simulink model "NBMS_MosfetSeq"  (R2026b)
settings: Solver=FixedStepDiscrete  StopTime=25  FixedStep=0.1
undefined symbols (not defined in the file): CAL_MOSFET_DISENG_THRSH, CAL_MOSFET_FEEDBACK, MosfetTime
settings Model: Creator=hp  LastModifiedBy=rathi
settings OptimizationCC: DefaultParameterBehavior=Inlined  DifferentSizesBufferReuse=on  EfficientTunableParamExpr=on  EnhancedBackFolding=on  OptimizationCustomize=off  OptimizeBlockOrder=speed  PassReuseOutputArgsAs=Individual arguments  RemoveInternalMemoryZeroInit=on  RemoveRootLevelIOMemoryZeroInit=on
settings DebuggingCC: ParameterTunabilityLossMsg=error
settings SFSimCC: MATLABDynamicMemAlloc=off
settings RTWCC: Description=Embedded Coder  GenCodeOnly=on  PackageGeneratedCodeAndArtifacts=on  SystemTargetFile=ert.tlc  TemplateMakefile=ert_default_tmf
settings CodeAppCC: ForceParamTrailComments=on  IgnoreCustomStorageClasses=off  InsertBlockDesc=on  OperatorAnnotations=on  SFDataObjDesc=on  SimulinkDataObjDesc=on
settings ERTTargetCC: DynamicArrayContainerType=coder::array  GenerateSampleERTMain=on
settings ConfigComp: DVDefectChecker=on  DVDetectOutOfBounds=on  DVHarnessSource=Signal Editor  DVModelReferenceHarness=on  DVTestSuiteOptimization=Auto

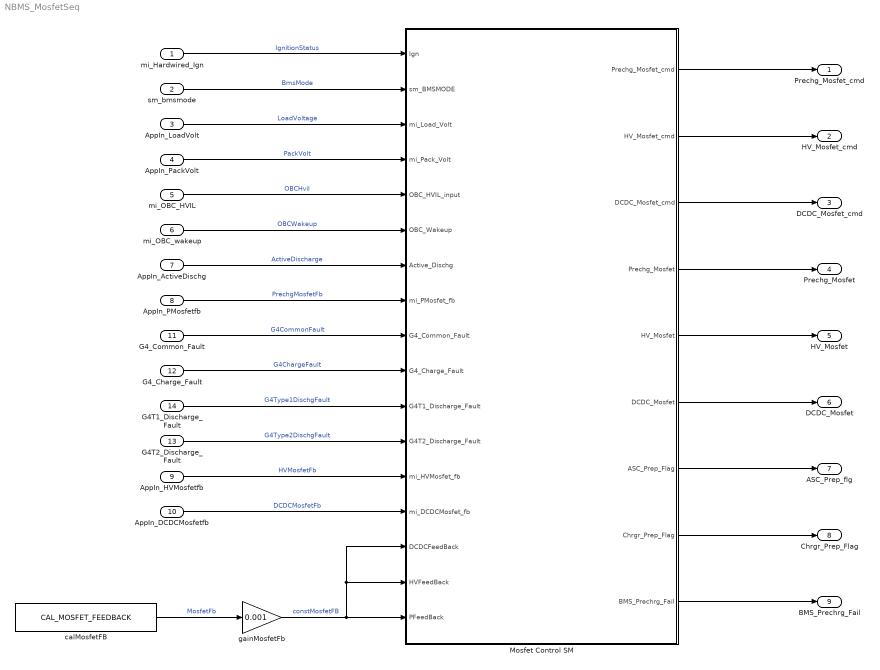
== system NBMS_MosfetSeq ==
  mi_Hardwired_Ign : Inport  OutDataTypeStr=boolean
  sm_bmsmode : Inport  Port=2  OutDataTypeStr=Enum: BMS_MODE_E
  AppIn_LoadVolt : Inport  Port=3  OutDataTypeStr=double
  AppIn_PackVolt : Inport  Port=4  OutDataTypeStr=double
  mi_OBC_HVIL : Inport  Port=5  OutDataTypeStr=boolean
  mi_OBC_wakeup : Inport  Port=6  OutDataTypeStr=Enum: OBC_E
  AppIn_ActiveDischg : Inport  Port=7  OutDataTypeStr=Enum: Active_DisChrg_E
  AppIn_PMosfetfb : Inport  Port=8  OutDataTypeStr=boolean
  AppIn_HVMosfetfb : Inport  Port=9  OutDataTypeStr=boolean
  AppIn_DCDCMosfetfb : Inport  Port=10  OutDataTypeStr=boolean
  G4_Common_Fault : Inport  Port=11  OutDataTypeStr=boolean
  G4_Charge_Fault : Inport  Port=12  OutDataTypeStr=boolean
  G4T2_Discharge_Fault : Inport  Port=13  OutDataTypeStr=boolean
  G4T1_Discharge_Fault : Inport  Port=14  OutDataTypeStr=boolean
  Mosfet Control SM : Stateflow chart  TreatAsAtomicUnit=on
      settings: PortSchema="{\"entries\":[{\"content\":{\"sides\":[{\"content\":{\"connectorIds\":[\"In1\",\"In2\",\"In3\",\"In4\",\"In5\",\"In6\",\"In7\",\"In13\",\"In14\",\"In15\",\"In16\",\"In17\",\"In12\",\"In11\",\"In8\",\"In9\",\"In10\"]},\"type\":\"ConnectorPlacement.EquallySpacedRectSide\",\"uuid\":\"999ebbd4-8031-46c1-80ce-b4c49c4d20a6\"},{\"content\":{\"connectorIds\":[\"Out1\",\"Out2\",\"Out3\",\"Out4\",\"Out5\",\"Out6\",\"Out7\",\"Out8\",\"Out9\"],\"side\":\"RIGHT\"},\"type\":\"ConnectorPlacement.EquallySpacedRectSide\",\"uuid\":\"fef7eb13-12a9-441d-9d81-95e69bfbb711\"},{\"content\":{\"side\":\"TOP\"},\"type\":\"ConnectorPlacement.EquallySpacedRectSide\",\"uuid\":\"5f60749b-759b-4b11-83fc-c9d02330dc93\"}]},\"type\":\"ConnectorPlacement.EquallySpacedConnector\",\"uuid\":\"de7edef1-d0c8-483b-a7d7-5a99a93b68ab\"}],\"packageUris\":[\"http://schema.mathworks.com/mf0/Connector/R2020b\"],\"version\":\"1.0\"}"
  calMosfetFB : Constant  Value=CAL_MOSFET_FEEDBACK
  gainMosfetFb : Gain  Gain=0.001  OutDataTypeStr=double
  Prechg_Mosfet_cmd : Outport  OutDataTypeStr=boolean
  HV_Mosfet_cmd : Outport  Port=2  OutDataTypeStr=boolean
  DCDC_Mosfet_cmd : Outport  Port=3  OutDataTypeStr=boolean
  Prechg_Mosfet : Outport  Port=4  OutDataTypeStr=Enum: BMS_PMosfet_STS_E
  HV_Mosfet : Outport  Port=5  OutDataTypeStr=Enum: BMS_HVMosfet_STS_E
  DCDC_Mosfet : Outport  Port=6  OutDataTypeStr=Enum: BMS_DCDCMosfet_STS_E
  ASC_Prep_flg : Outport  Port=7  OutDataTypeStr=boolean
  Chrgr_Prep_Flag : Outport  Port=8  OutDataTypeStr=boolean
  BMS_Prechrg_Fail : Outport  Port=9  OutDataTypeStr=boolean
  wires:
  mi_Hardwired_Ign/1 -> Mosfet Control SM/1(Ign)  "IgnitionStatus"
  sm_bmsmode/1 -> Mosfet Control SM/2(sm_BMSMODE)  "BmsMode"
  AppIn_LoadVolt/1 -> Mosfet Control SM/3(mi_Load_Volt)  "LoadVoltage"
  AppIn_PackVolt/1 -> Mosfet Control SM/4(mi_Pack_Volt)  "PackVolt"
  mi_OBC_HVIL/1 -> Mosfet Control SM/5(OBC_HVIL_input)  "OBCHvil"
  mi_OBC_wakeup/1 -> Mosfet Control SM/6(OBC_Wakeup)  "OBCWakeup"
  AppIn_ActiveDischg/1 -> Mosfet Control SM/7(Active_Dischg)  "ActiveDischarge"
  Mosfet Control SM/3(DCDC_Mosfet_cmd) -> DCDC_Mosfet_cmd/1
  Mosfet Control SM/2(HV_Mosfet_cmd) -> HV_Mosfet_cmd/1
  Mosfet Control SM/1(Prechg_Mosfet_cmd) -> Prechg_Mosfet_cmd/1
  Mosfet Control SM/4(Prechg_Mosfet) -> Prechg_Mosfet/1
  Mosfet Control SM/5(HV_Mosfet) -> HV_Mosfet/1
  Mosfet Control SM/6(DCDC_Mosfet) -> DCDC_Mosfet/1
  Mosfet Control SM/7(ASC_Prep_Flag) -> ASC_Prep_flg/1
  calMosfetFB/1 -> gainMosfetFb/1  "MosfetFb"
  gainMosfetFb/1 -> Mosfet Control SM/8(DCDCFeedBack), Mosfet Control SM/9(HVFeedBack), Mosfet Control SM/10(PFeedBack)  "constMosfetFB"
  AppIn_PMosfetfb/1 -> Mosfet Control SM/13(mi_PMosfet_fb)  "PrechgMosfetFb"
  AppIn_HVMosfetfb/1 -> Mosfet Control SM/12(mi_HVMosfet_fb)  "HVMosfetFb"
  AppIn_DCDCMosfetfb/1 -> Mosfet Control SM/11(mi_DCDCMosfet_fb)  "DCDCMosfetFb"
  G4_Common_Fault/1 -> Mosfet Control SM/14(G4_Common_Fault)  "G4CommonFault"
  G4_Charge_Fault/1 -> Mosfet Control SM/15(G4_Charge_Fault)  "G4ChargeFault"
  G4T2_Discharge_Fault/1 -> Mosfet Control SM/17(G4T2_Discharge_Fault)  "G4Type2DischgFault"
  G4T1_Discharge_Fault/1 -> Mosfet Control SM/16(G4T1_Discharge_Fault)  "G4Type1DischgFault"
  Mosfet Control SM/8(Chrgr_Prep_Flag) -> Chrgr_Prep_Flag/1
  Mosfet Control SM/9(BMS_Prechrg_Fail) -> BMS_Prechrg_Fail/1

== stateflow chart NBMS_MosfetSeq/Mosfet Control SM ==
  state DEFAULT
    state DEF
    state STANDBY
      state DEFAULT
        HV_Mosfet_cmd = false;
      state OpenHVMosfet
        HV_Mosfet = BMS_HVMosfet_STS_E.HV_DISCONNECTED;
      state OpenDCDCMosfet
        en:
        DCDC_Mosfet_cmd = false;
        DCDC_Mosfet = BMS_DCDCMosfet_STS_E.DCDC_DISCONNECTED;
      (default) -> DEFAULT.STANDBY.DEFAULT : {NA = false;}
      DEFAULT.STANDBY.DEFAULT -> DEFAULT.STANDBY.OpenHVMosfet : [duration(mi_HVMosfet_fb==0)>=HVFeedBack]
      DEFAULT.STANDBY.OpenHVMosfet -> DEFAULT.STANDBY.OpenDCDCMosfet : [Active_Dischg == Active_DisChrg_E.Completed || ...
          | sm_BMSMODE == BMS_MODE_E.BMS_SLEEP]
    state No_Action
      NA = true;
      state CloseDCDC
        DCDC_Mosfet_cmd = true;
        DCDC_Mosfet = BMS_DCDCMosfet_STS_E.DCDC_CONNECTED;
      state OpenDCDC
        DCDC_Mosfet_cmd = false;
        DCDC_Mosfet = BMS_DCDCMosfet_STS_E.DCDC_DISCONNECTED;
      (default) -> DEFAULT.No_Action.CloseDCDC
      DEFAULT.No_Action.CloseDCDC -> DEFAULT.No_Action.OpenDCDC : [sm_BMSMODE == BMS_MODE_E.BMS_CHARGE && Ign == false]
      DEFAULT.No_Action.OpenDCDC -> DEFAULT.No_Action.CloseDCDC : [Ign == true]
    state G4CommonFault
      state OnFaultDetection
        state OpenHVMosfet
          en:
          Prechg_Mosfet = BMS_PMosfet_STS_E.PDISCONNECTED;
          HV_Mosfet = BMS_HVMosfet_STS_E.HV_DISCONNECTED;
          Prechg_Mosfet_cmd = false;
          HV_Mosfet_cmd = false;
        state Def
          en:
          count1 = 0;
          du:
          count1 = count1 + 100;
        (default) -> DEFAULT.G4CommonFault.OnFaultDetection.Def
        DEFAULT.G4CommonFault.OnFaultDetection.Def -> DEFAULT.G4CommonFault.OnFaultDetection.OpenHVMosfet : [count1>=CAL_MOSFET_DISENG_THRSH]
            | {NA = false; Chrgr_Prep_Flag = false; ASC_Prep_Flag = false;}
      state BMS_Sleep
        en:
        Prechg_Mosfet = BMS_PMosfet_STS_E.PDISCONNECTED;
        HV_Mosfet = BMS_HVMosfet_STS_E.HV_DISCONNECTED;
        DCDC_Mosfet = BMS_DCDCMosfet_STS_E.DCDC_DISCONNECTED;
        Prechg_Mosfet_cmd = false;
        HV_Mosfet_cmd = false;
        DCDC_Mosfet_cmd = false;
        BMS_Prechrg_Fail = false;
      (default) -> DEFAULT.G4CommonFault.OnFaultDetection
      DEFAULT.G4CommonFault.OnFaultDetection -> DEFAULT.G4CommonFault.BMS_Sleep : [(sm_BMSMODE == BMS_MODE_E.BMS_FAULT && Ign == false && ...
          | Active_Dischg == Active_DisChrg_E.Completed) || ...
          | sm_BMSMODE == BMS_MODE_E.BMS_SLEEP]
    state G4Typ1DischgFault
      state OnFaultDetection
        state OpenHVMosfet
          en:
          Prechg_Mosfet = BMS_PMosfet_STS_E.PDISCONNECTED;
          HV_Mosfet = BMS_HVMosfet_STS_E.HV_DISCONNECTED;
          Prechg_Mosfet_cmd = false;
          HV_Mosfet_cmd = false;
        state Def
          en:
          count = 0;
          du:
          count = count + 100;
        (default) -> DEFAULT.G4Typ1DischgFault.OnFaultDetection.Def
        DEFAULT.G4Typ1DischgFault.OnFaultDetection.Def -> DEFAULT.G4Typ1DischgFault.OnFaultDetection.OpenHVMosfet : [count>=CAL_MOSFET_DISENG_THRSH]
            | {NA = false; ASC_Prep_Flag = false;}
      state BMS_Sleep
        en:
        Prechg_Mosfet = BMS_PMosfet_STS_E.PDISCONNECTED;
        HV_Mosfet = BMS_HVMosfet_STS_E.HV_DISCONNECTED;
        DCDC_Mosfet = BMS_DCDCMosfet_STS_E.DCDC_DISCONNECTED;
        Prechg_Mosfet_cmd = false;
        HV_Mosfet_cmd = false;
        DCDC_Mosfet_cmd = false;
        BMS_Prechrg_Fail = false;
      (default) -> DEFAULT.G4Typ1DischgFault.OnFaultDetection
      DEFAULT.G4Typ1DischgFault.OnFaultDetection -> DEFAULT.G4Typ1DischgFault.BMS_Sleep : [(sm_BMSMODE == BMS_MODE_E.BMS_FAULT && Ign == false && ...
          | Active_Dischg == Active_DisChrg_E.Completed) || ...
          | sm_BMSMODE == BMS_MODE_E.BMS_SLEEP]
    state G4Typ2DischgFault
      state OnFaultDetection
        state OpenHVMosfet
          en:
          Prechg_Mosfet = BMS_PMosfet_STS_E.PDISCONNECTED;
          HV_Mosfet = BMS_HVMosfet_STS_E.HV_DISCONNECTED;
          DCDC_Mosfet = BMS_DCDCMosfet_STS_E.DCDC_DISCONNECTED;
          Prechg_Mosfet_cmd = false;
          HV_Mosfet_cmd = false;
          DCDC_Mosfet_cmd = false;
        state Def
          en:
          count2 = 0;
          du:
          count2 = count2 + 100;
        (default) -> DEFAULT.G4Typ2DischgFault.OnFaultDetection.Def
        DEFAULT.G4Typ2DischgFault.OnFaultDetection.Def -> DEFAULT.G4Typ2DischgFault.OnFaultDetection.OpenHVMosfet : [count2>=CAL_MOSFET_DISENG_THRSH]
            | {NA = false; ASC_Prep_Flag = false;}
      state BMS_Sleep
        en:
        Prechg_Mosfet = BMS_PMosfet_STS_E.PDISCONNECTED;
        HV_Mosfet = BMS_HVMosfet_STS_E.HV_DISCONNECTED;
        DCDC_Mosfet = BMS_DCDCMosfet_STS_E.DCDC_DISCONNECTED;
        Prechg_Mosfet_cmd = false;
        HV_Mosfet_cmd = false;
        DCDC_Mosfet_cmd = false;
        BMS_Prechrg_Fail = false;
      (default) -> DEFAULT.G4Typ2DischgFault.OnFaultDetection
      DEFAULT.G4Typ2DischgFault.OnFaultDetection -> DEFAULT.G4Typ2DischgFault.BMS_Sleep : [(sm_BMSMODE == BMS_MODE_E.BMS_FAULT && Ign == false && ...
          | Active_Dischg == Active_DisChrg_E.Completed) || ...
          | sm_BMSMODE == BMS_MODE_E.BMS_SLEEP]
    state G4ChargeFault
      state OnFaultDetection
        state OpenHVMosfet
          en:
          Prechg_Mosfet = BMS_PMosfet_STS_E.PDISCONNECTED;
          HV_Mosfet = BMS_HVMosfet_STS_E.HV_DISCONNECTED;
          Prechg_Mosfet_cmd = false;
          HV_Mosfet_cmd = false;
        state Def
          en:
          count3 = 0;
          du:
          count3 = count3 + 100;
        (default) -> DEFAULT.G4ChargeFault.OnFaultDetection.Def
        DEFAULT.G4ChargeFault.OnFaultDetection.Def -> DEFAULT.G4ChargeFault.OnFaultDetection.OpenHVMosfet : [count3>=CAL_MOSFET_DISENG_THRSH]
            | {NA = false; Chrgr_Prep_Flag = false;}
      state BMS_Sleep
        en:
        Prechg_Mosfet = BMS_PMosfet_STS_E.PDISCONNECTED;
        HV_Mosfet = BMS_HVMosfet_STS_E.HV_DISCONNECTED;
        DCDC_Mosfet = BMS_DCDCMosfet_STS_E.DCDC_DISCONNECTED;
        Prechg_Mosfet_cmd = false;
        HV_Mosfet_cmd = false;
        DCDC_Mosfet_cmd = false;
        BMS_Prechrg_Fail = false;
      (default) -> DEFAULT.G4ChargeFault.OnFaultDetection
      DEFAULT.G4ChargeFault.OnFaultDetection -> DEFAULT.G4ChargeFault.BMS_Sleep : [(sm_BMSMODE == BMS_MODE_E.BMS_FAULT && Ign == false && ...
          | Active_Dischg == Active_DisChrg_E.Completed) || ...
          | sm_BMSMODE == BMS_MODE_E.BMS_SLEEP]
    (default) -> DEF : {Prechg_Mosfet_cmd = false;HV_Mosfet_cmd = false;
        | DCDC_Mosfet_cmd = false;
        | Prechg_Mosfet = BMS_PMosfet_STS_E.PDISCONNECTED;
        | HV_Mosfet = BMS_HVMosfet_STS_E.HV_DISCONNECTED;
        | DCDC_Mosfet = BMS_DCDCMosfet_STS_E.DCDC_DISCONNECTED;
        | BMS_Prechrg_Fail = false;
        | ASC_Prep_Flag = false;NA = false;}
    (junction 390) -> STANDBY : [[(Ign == true && OBC_HVIL_input == true) || ...
        | Ign == false || OBC_Wakeup ~= OBC_E.Wake_Up]]
    No_Action -> (junction 390) [order 1] : [sm_BMSMODE == BMS_MODE_E.BMS_STANDBY]
    STANDBY -> (junction 494) [order 3]
    STANDBY -> (junction 488) [order 2] : [G4T1_Discharge_Fault == true]{ASC_Prep_Flag = true;}
    STANDBY -> G4CommonFault [order 1] : [G4_Common_Fault == true]
        | {ASC_Prep_Flag = true; Chrgr_Prep_Flag = true;}
    (junction 494) -> (junction 497) [order 2] : [G4_Charge_Fault == true]
        | {Chrgr_Prep_Flag = true;}
    No_Action -> (junction 494) [order 4]
    (junction 497) -> G4ChargeFault
    (junction 494) -> G4Typ2DischgFault [order 1] : [G4T2_Discharge_Fault == true]
        | {ASC_Prep_Flag = true;}
    No_Action -> G4CommonFault [order 2] : [G4_Common_Fault == true]
        | {ASC_Prep_Flag = true; Chrgr_Prep_Flag = true;}
    No_Action -> G4Typ1DischgFault [order 3] : [G4T1_Discharge_Fault == true]
        | {ASC_Prep_Flag = true;}
    (junction 488) -> G4Typ1DischgFault
    G4Typ1DischgFault -> G4Typ2DischgFault : [G4T2_Discharge_Fault == true]
        | {ASC_Prep_Flag = true;}
    (junction 358) -> G4Typ2DischgFault
  state Mosfet_Sequence
    state CLOSING_SEQ
      state ClosePrechgMosfet
        Prechg_Mosfet_cmd = true;
      state CheckPrechgVolt
      state PrechgVoltFailure
        en:
        BMS_Prechrg_Fail = true;
        Prechg_Mosfet_cmd = false;
      state CloseHVMosfet
        HV_Mosfet_cmd = true;
      state CloseDCDCMosfet
        DCDC_Mosfet_cmd = true;
      state OpenPrechgMosfet
        Prechg_Mosfet_cmd = false;
      state Positiveclosed
        HV_Mosfet = BMS_HVMosfet_STS_E.HV_CONNECTED;
      state OpenDCDCMosfetIgOff
        state CloseDCDC
          DCDC_Mosfet_cmd = true;
          DCDC_Mosfet = BMS_DCDCMosfet_STS_E.DCDC_CONNECTED;
        state OpenDCDC
          DCDC_Mosfet_cmd = false;
          DCDC_Mosfet = BMS_DCDCMosfet_STS_E.DCDC_DISCONNECTED;
        (default) -> Mosfet_Sequence.CLOSING_SEQ.OpenDCDCMosfetIgOff.OpenDCDC
        Mosfet_Sequence.CLOSING_SEQ.OpenDCDCMosfetIgOff.CloseDCDC -> Mosfet_Sequence.CLOSING_SEQ.OpenDCDCMosfetIgOff.OpenDCDC : [Ign == false]
        Mosfet_Sequence.CLOSING_SEQ.OpenDCDCMosfetIgOff.OpenDCDC -> Mosfet_Sequence.CLOSING_SEQ.OpenDCDCMosfetIgOff.CloseDCDC : [Ign == true]
      (default) -> Mosfet_Sequence.CLOSING_SEQ.ClosePrechgMosfet
      Mosfet_Sequence.CLOSING_SEQ.ClosePrechgMosfet -> Mosfet_Sequence.CLOSING_SEQ.CheckPrechgVolt : [duration(mi_PMosfet_fb==1)>=PFeedBack]
          | {Prechg_Mosfet = BMS_PMosfet_STS_E.PCONNECTED;}
      Mosfet_Sequence.CLOSING_SEQ.CheckPrechgVolt -> Mosfet_Sequence.CLOSING_SEQ.PrechgVoltFailure [order 2] : [mi_Load_Volt/mi_Pack_Volt < 0.95 && after(MosfetTime,msec)]
      Mosfet_Sequence.CLOSING_SEQ.CheckPrechgVolt -> Mosfet_Sequence.CLOSING_SEQ.CloseHVMosfet [order 1] : [mi_Load_Volt/mi_Pack_Volt >= 0.95]
      Mosfet_Sequence.CLOSING_SEQ.CloseHVMosfet -> CloseDCDCMosfet : [duration(mi_HVMosfet_fb==1)>=HVFeedBack]
          | {HV_Mosfet = BMS_HVMosfet_STS_E.HV_CONNECT_PENDING;}
      CloseDCDCMosfet -> Mosfet_Sequence.CLOSING_SEQ.OpenPrechgMosfet : [duration(mi_DCDCMosfet_fb==1)>=DCDCFeedBack]
          | {DCDC_Mosfet = BMS_DCDCMosfet_STS_E.DCDC_CONNECTED;}
      Mosfet_Sequence.CLOSING_SEQ.OpenPrechgMosfet -> Mosfet_Sequence.CLOSING_SEQ.Positiveclosed : [duration(mi_PMosfet_fb==0)>=PFeedBack]
          | {Prechg_Mosfet = BMS_PMosfet_STS_E.PDISCONNECTED;}
      Mosfet_Sequence.CLOSING_SEQ.Positiveclosed -> OpenDCDCMosfetIgOff : [sm_BMSMODE == BMS_MODE_E.BMS_CHARGE && Ign == false && Active_Dischg == Active_DisChrg_E.Completed]
    state CLOSING_SEQ_CHRG
      state ClosePrechgMosfet
        Prechg_Mosfet_cmd = true;
      state CheckPrechgVolt
      state PrechgVoltFailure
        en:
        BMS_Prechrg_Fail = true;
        Prechg_Mosfet_cmd = false;
      state CloseHVMosfet
        HV_Mosfet_cmd = true;
      state OpenDCDCMosfet
        DCDC_Mosfet_cmd = false;
      state OpenPrechgMosfet
        Prechg_Mosfet_cmd = false;
      state Positiveclosed
        HV_Mosfet = BMS_HVMosfet_STS_E.HV_CONNECTED;
      state CloseDCDCMosfetIgOn
        state CloseDCDC
          DCDC_Mosfet_cmd = true;
          DCDC_Mosfet = BMS_DCDCMosfet_STS_E.DCDC_CONNECTED;
        state OpenDCDC
          DCDC_Mosfet_cmd = false;
          DCDC_Mosfet = BMS_DCDCMosfet_STS_E.DCDC_DISCONNECTED;
        (default) -> Mosfet_Sequence.CLOSING_SEQ_CHRG.CloseDCDCMosfetIgOn.CloseDCDC
        Mosfet_Sequence.CLOSING_SEQ_CHRG.CloseDCDCMosfetIgOn.CloseDCDC -> Mosfet_Sequence.CLOSING_SEQ_CHRG.CloseDCDCMosfetIgOn.OpenDCDC : [Ign == false]
        Mosfet_Sequence.CLOSING_SEQ_CHRG.CloseDCDCMosfetIgOn.OpenDCDC -> Mosfet_Sequence.CLOSING_SEQ_CHRG.CloseDCDCMosfetIgOn.CloseDCDC : [Ign == true]
      (default) -> Mosfet_Sequence.CLOSING_SEQ_CHRG.ClosePrechgMosfet
      Mosfet_Sequence.CLOSING_SEQ_CHRG.ClosePrechgMosfet -> Mosfet_Sequence.CLOSING_SEQ_CHRG.CheckPrechgVolt : [duration(mi_PMosfet_fb==1)>=PFeedBack]
          | {Prechg_Mosfet = BMS_PMosfet_STS_E.PCONNECTED;}
      Mosfet_Sequence.CLOSING_SEQ_CHRG.CheckPrechgVolt -> Mosfet_Sequence.CLOSING_SEQ_CHRG.PrechgVoltFailure [order 2] : [mi_Load_Volt/mi_Pack_Volt < 0.95 && after(MosfetTime,msec)]
      Mosfet_Sequence.CLOSING_SEQ_CHRG.CheckPrechgVolt -> Mosfet_Sequence.CLOSING_SEQ_CHRG.CloseHVMosfet [order 1] : [mi_Load_Volt/mi_Pack_Volt >= 0.95]
      Mosfet_Sequence.CLOSING_SEQ_CHRG.CloseHVMosfet -> Mosfet_Sequence.CLOSING_SEQ_CHRG.OpenDCDCMosfet : [duration(mi_HVMosfet_fb==1)>=HVFeedBack]
          | {HV_Mosfet = BMS_HVMosfet_STS_E.HV_CONNECT_PENDING;}
      Mosfet_Sequence.CLOSING_SEQ_CHRG.OpenDCDCMosfet -> Mosfet_Sequence.CLOSING_SEQ_CHRG.OpenPrechgMosfet : [duration(mi_DCDCMosfet_fb==0)>=DCDCFeedBack]
          | {DCDC_Mosfet = BMS_DCDCMosfet_STS_E.DCDC_DISCONNECTED;}
      Mosfet_Sequence.CLOSING_SEQ_CHRG.OpenPrechgMosfet -> Mosfet_Sequence.CLOSING_SEQ_CHRG.Positiveclosed : [duration(mi_PMosfet_fb==0)>=PFeedBack]
          | {Prechg_Mosfet = BMS_PMosfet_STS_E.PDISCONNECTED;}
      Mosfet_Sequence.CLOSING_SEQ_CHRG.Positiveclosed -> CloseDCDCMosfetIgOn : [sm_BMSMODE == BMS_MODE_E.BMS_CHARGE && Ign == true]
  (default) -> DEFAULT
  DEFAULT -> CLOSING_SEQ [order 1] : [(Ign == true) && ...
      | (sm_BMSMODE == BMS_MODE_E.BMS_DISCHARGE || ...
      | sm_BMSMODE == BMS_MODE_E.BMS_CHARGE) && NA == false]
  Mosfet_Sequence -> (junction 390) [order 1] : [duration(sm_BMSMODE == BMS_MODE_E.BMS_STANDBY) >= 0.2]
  Mosfet_Sequence -> No_Action [order 2] : [HV_Mosfet == BMS_HVMosfet_STS_E.HV_CONNECTED && ...
      | DCDC_Mosfet == BMS_DCDCMosfet_STS_E.DCDC_CONNECTED && ...
      | ((hasChangedTo(sm_BMSMODE, BMS_MODE_E.BMS_DISCHARGE)) || ...
      | (hasChangedTo(sm_BMSMODE, BMS_MODE_E.BMS_CHARGE)))]
  DEFAULT -> CLOSING_SEQ_CHRG [order 2] : [Ign == false && sm_BMSMODE == BMS_MODE_E.BMS_CHARGE && NA == false]
  Mosfet_Sequence -> G4CommonFault [order 6] : [G4_Common_Fault == true || BMS_Prechrg_Fail == true]
      | {ASC_Prep_Flag = true; Chrgr_Prep_Flag = true;}
  Mosfet_Sequence -> G4Typ1DischgFault [order 4] : [G4T1_Discharge_Fault == true]{ASC_Prep_Flag = true;}
  Mosfet_Sequence -> (junction 358) [order 5] : [G4T2_Discharge_Fault == true]{ASC_Prep_Flag = true;}
  Mosfet_Sequence -> G4ChargeFault [order 3] : [G4_Charge_Fault == true]{Chrgr_Prep_Flag = true;}
  data: Ign input; sm_BMSMODE input; mi_Load_Volt input; mi_Pack_Volt input; OBC_HVIL_input input; OBC_Wakeup input; Prechg_Mosfet_cmd output; HV_Mosfet_cmd output; Active_Dischg input; DCDC_Mosfet_cmd output; Prechg_Mosfet output; HV_Mosfet output; DCDC_Mosfet output; NA local; ASC_Prep_Flag output; DCDCFeedBack input; HVFeedBack input; PFeedBack input; mi_DCDCMosfet_fb input; mi_HVMosfet_fb input; mi_PMosfet_fb input; CAL_MOSFET_DISENG_THRSH parameter; count1 local; count local; Chrgr_Prep_Flag output; G4_Common_Fault input; G4_Charge_Fault input; G4T1_Discharge_Fault input; G4T2_Discharge_Fault input; MosfetTime parameter; count3 local; count2 local; BMS_Prechrg_Fail output
